simulink model "cable_driven_parallel_robot"  (R2023a)
settings: Solver=ode3  StartTime=0.0  StopTime=100  FixedStep=0.01  RelTol=1e-3
values from neighbouring files (symbols this model uses):
  cable_length = 1.2    [Model_Info.m]
  g = 9.81    [Model_Info.m]
  MP_H = 2    [Model_Info.m]
  MP_init_X = 0    [Model_Info.m]
  MP_init_Y = 0    [Model_Info.m]
  MP_init_Z = cable_length + (MP_H/2)    (= 2.2)    [Model_Info.m]
  MP_Ix = (MP_m/12)*(MP_W^2+MP_H^2)    (= 6.66666666667e-05)    [Model_Info.m]
  MP_Iy = (MP_m/12)*(MP_L^2+MP_H^2)    (= 6.66666666667e-05)    [Model_Info.m]
  MP_Iz = (MP_m/12)*(MP_L^2+MP_W^2)    (= 6.66666666667e-05)    [Model_Info.m]
  MP_L = 2    [Model_Info.m]
  MP_m = 0.0001    [Model_Info.m]
  MP_W = 2    [Model_Info.m]
  MR_init_X_L1 = -(MP_L/2)    (= -1)    [Model_Info.m]
  MR_init_X_L2 = (MP_L/2)    (= 1)    [Model_Info.m]
  MR_init_X_L3 = (MP_L/2)    (= 1)    [Model_Info.m]
  MR_init_X_L4 = -(MP_L/2)    (= -1)    [Model_Info.m]
  MR_init_Y_L1 = -(MP_W/2)    (= -1)    [Model_Info.m]
  MR_init_Y_L2 = -(MP_W/2)    (= -1)    [Model_Info.m]
  MR_init_Y_L3 = (MP_W/2)    (= 1)    [Model_Info.m]
  MR_init_Y_L4 = (MP_W/2)    (= 1)    [Model_Info.m]
  MR_init_Yaw_L1 = pi    (= 3.14159265359)    [Model_Info.m]
  MR_init_Yaw_L2 = 0    [Model_Info.m]
  MR_init_Yaw_L3 = 0    [Model_Info.m]
  MR_init_Yaw_L4 = pi    (= 3.14159265359)    [Model_Info.m]
  MR_Jr = (MR_m/12)*(MR_L^2+MR_W^2)    (= 0.333333333333)    [Model_Info.m]
  MR_m = 0.5    [Model_Info.m]
  MR_r = 2    [Model_Info.m]
  MR_WT = 2    [Model_Info.m]
  QR_Ax = 0.25*0    (= 0)    [Model_Info.m]
  QR_Ay = 0.25*0    (= 0)    [Model_Info.m]
  QR_Az = 0.25*0    (= 0)    [Model_Info.m]
  QR_b = 1.14*1e-7    (= 1.14e-07)    [Model_Info.m]
  QR_Ixx = 4.856*1e-3    (= 0.004856)    [Model_Info.m]
  QR_Iyy = 4.856*1e-3    (= 0.004856)    [Model_Info.m]
  QR_Izz = 8.801*1e-3    (= 0.008801)    [Model_Info.m]
  QR_K = 2.980*1e-6    (= 2.98e-06)    [Model_Info.m]
  QR_l = 0.225    [Model_Info.m]
  QR_m = 0.468    [Model_Info.m]
  QR_x0_U1 = -(MP_L/2)    (= -1)    [Model_Info.m]
  QR_x0_U2 = (MP_L/2)    (= 1)    [Model_Info.m]
  QR_x0_U3 = (MP_L/2)    (= 1)    [Model_Info.m]
  QR_x0_U4 = -(MP_L/2)    (= -1)    [Model_Info.m]
  QR_y0_U1 = -(MP_W/2)    (= -1)    [Model_Info.m]
  QR_y0_U2 = -(MP_W/2)    (= -1)    [Model_Info.m]
  QR_y0_U3 = (MP_W/2)    (= 1)    [Model_Info.m]
  QR_y0_U4 = (MP_W/2)    (= 1)    [Model_Info.m]
  QR_z0_U1 = 2*cable_length+(MP_H)    (= 4.4)    [Model_Info.m]
  QR_z0_U2 = 2*cable_length+(MP_H)    (= 4.4)    [Model_Info.m]
  QR_z0_U3 = 2*cable_length+(MP_H)    (= 4.4)    [Model_Info.m]
  QR_z0_U4 = 2*cable_length+(MP_H)    (= 4.4)    [Model_Info.m]
(part 10 of 12)

== matlab function cable_driven_parallel_robot/Target Wrench-Jacobian matrix/QuadRotor U1/Force Generator/QuadCopter Model ==
  data: vx input; x_ddot output size=1; vy input; vz input; phidot input; thetadot input; psidot input; y_ddot output size=1; z_ddot output size=1; phi input; theta input; psi input; constants input
function [x_ddot,y_ddot,z_ddot] = fcn(vx,vy,vz,phidot,thetadot,psidot, phi,theta,psi,constants)
m = constants(1);
g = constants(2);
Ixx = constants(3);
Iyy = constants(4);
Izz = constants(5);
l = constants(6);
K = constants(7);
b = constants(8);
Ax = constants(9);
Ay = constants(10);
Az = constants(11);
omega1 = constants(12);
omega2 = constants(13);
omega3 = constants(14);
omega4 = constants(15);
Tx = constants(16);
Ty = constants(17);
Tz = constants(18);
% x_ddot = (K*omega1^2*sin(phi)*sin(psi) - Ax*vx + K*omega2^2*sin(phi)*sin(psi) + K*omega3^2*sin(phi)*sin(psi) + K*omega4^2*sin(phi)*sin(psi) + K*omega1^2*cos(phi)*cos(psi)*sin(theta) + K*omega2^2*cos(phi)*cos(psi)*sin(theta) + K*omega3^2*cos(phi)*cos(psi)*sin(theta) + K*omega4^2*cos(phi)*cos(psi)*sin(theta))/m;
% y_ddot = -(Ay*vy + K*omega1^2*cos(psi)*sin(phi) + K*omega2^2*cos(psi)*sin(phi) + K*omega3^2*cos(psi)*sin(phi) + K*omega4^2*cos(psi)*sin(phi) - K*omega1^2*cos(phi)*sin(psi)*sin(theta) - K*omega2^2*cos(phi)*sin(psi)*sin(theta) - K*omega3^2*cos(phi)*sin(psi)*sin(theta) - K*omega4^2*cos(phi)*sin(psi)*sin(theta))/m;
% z_ddot = (K*cos(phi)*cos(theta)*omega1^2 + K*cos(phi)*cos(theta)*omega2^2 + K*cos(phi)*cos(theta)*omega3^2 + K*cos(phi)*cos(theta)*omega4^2 - Az*vz - g*m)/m;
% phi_ddot = (2*Ixx*Iyy*b*omega1^2*sin(theta) - 2*Ixx*Iyy*b*omega2^2*sin(theta) + 2*Ixx*Iyy*b*omega3^2*sin(theta) - 2*Ixx*Iyy*b*omega4^2*sin(theta) + 2*Iyy^3*psidot^2*cos(phi)*cos(theta)^4*sin(phi)^3 - 2*Iyy^3*psidot^2*cos(phi)*cos(theta)^4*sin(phi)^5 - 2*Iyy^3*psidot*thetadot*cos(theta)^3*sin(phi)^2 + 2*Iyy^3*psidot*thetadot*cos(theta)^3*sin(phi)^4 - 2*Iyy^3*psidot^2*cos(phi)^3*cos(theta)^4*sin(phi)^3 - Iyy^3*thetadot^2*sin(2*phi)*cos(theta)^2*sin(phi)^2 + Iyy^3*thetadot^2*sin(2*phi)*cos(theta)^2*sin(phi)^4 - Ixx*Iyy^2*thetadot^2*sin(2*phi)*sin(theta)^2 - 2*Iyy^2*K*l*omega2^2*cos(theta)^2*sin(phi)^2 + 2*Iyy^2*K*l*omega2^2*cos(theta)^2*sin(phi)^4 + 2*Iyy^2*K*l*omega4^2*cos(theta)^2*sin(phi)^2 - 2*Iyy^2*K*l*omega4^2*cos(theta)^2*sin(phi)^4 + 2*Ixx*Iyy^2*thetadot^2*cos(phi)*sin(phi)*sin(theta)^2 - 2*Ixx*Iyy*b*omega1^2*sin(phi)^2*sin(theta) + 2*Ixx*Iyy*b*omega2^2*sin(phi)^2*sin(theta) - 2*Ixx*Iyy*b*omega3^2*sin(phi)^2*sin(theta) + 2*Ixx*Iyy*b*omega4^2*sin(phi)^2*sin(theta) + 2*Ixx*Izz*b*omega1^2*sin(phi)^2*sin(theta) - 2*Ixx*Izz*b*omega2^2*sin(phi)^2*sin(theta) + 2*Ixx*Izz*b*omega3^2*sin(phi)^2*sin(theta) - 2*Ixx*Izz*b*omega4^2*sin(phi)^2*sin(theta) - 2*Ixx*Iyy^2*psidot*thetadot*cos(theta)*sin(theta)^2 + 2*Ixx^2*Iyy*psidot*thetadot*cos(theta)*sin(theta)^2 + 2*Ixx*Iyy^2*psidot*thetadot*sin(2*theta)*sin(theta) - 2*Ixx^2*Iyy*psidot*thetadot*sin(2*theta)*sin(theta) - 2*Iyy*Izz^2*psidot^2*cos(phi)^3*cos(theta)^4*sin(phi) - 2*Iyy^2*Izz*psidot^2*cos(phi)*cos(theta)^4*sin(phi)^3 + 2*Iyy^2*Izz*psidot^2*cos(phi)^3*cos(theta)^4*sin(phi) - 2*Iyy*Izz^2*psidot^2*cos(phi)*cos(theta)^4*sin(phi)^5 + 4*Iyy^2*Izz*psidot^2*cos(phi)*cos(theta)^4*sin(phi)^5 - 2*Ixx*Iyy^2*thetadot^2*cos(phi)*sin(phi)^3*sin(theta)^2 - 2*Ixx*Izz^2*thetadot^2*cos(phi)*sin(phi)^3*sin(theta)^2 + Ixx*Iyy*Izz*thetadot^2*sin(2*phi)*sin(theta)^2 + 6*Iyy^3*psidot*thetadot*cos(phi)^2*cos(theta)^3*sin(phi)^2 - 4*Iyy^3*psidot*thetadot*cos(phi)^2*cos(theta)^3*sin(phi)^4 - 4*Iyy^3*psidot*thetadot*cos(phi)^4*cos(theta)^3*sin(phi)^2 + 2*Iyy*Izz^2*psidot*thetadot*cos(phi)^2*cos(theta)^3 - 2*Iyy^2*Izz*psidot*thetadot*cos(phi)^2*cos(theta)^3 - 4*Iyy*Izz^2*psidot*thetadot*cos(phi)^4*cos(theta)^3 + 4*Iyy^2*Izz*psidot*thetadot*cos(phi)^4*cos(theta)^3 + 2*Ixx*Iyy^2*psidot*thetadot*cos(theta)^3*sin(phi)^2 - 2*Ixx*Iyy^2*psidot*thetadot*cos(theta)^3*sin(phi)^4 + 2*Iyy^2*Izz*psidot*thetadot*cos(theta)^3*sin(phi)^2 + 2*Iyy*Izz^2*psidot*thetadot*cos(theta)^3*sin(phi)^4 - 4*Iyy^2*Izz*psidot*thetadot*cos(theta)^3*sin(phi)^4 - 2*Ixx*Iyy*K*l*omega2^2*sin(theta)^2 + 2*Ixx*Iyy*K*l*omega4^2*sin(theta)^2 + Iyy^3*thetadot^2*sin(2*phi)*cos(phi)^2*cos(theta)^2*sin(phi)^2 - 2*Iyy*Izz^2*psidot^2*cos(phi)^3*cos(theta)^4*sin(phi)^3 + 4*Iyy^2*Izz*psidot^2*cos(phi)^3*cos(theta)^4*sin(phi)^3 + Iyy*Izz^2*thetadot^2*sin(2*phi)*cos(phi)^2*cos(theta)^2 - Iyy^2*Izz*thetadot^2*sin(2*phi)*cos(phi)^2*cos(theta)^2 + Iyy^2*Izz*thetadot^2*sin(2*phi)*cos(theta)^2*sin(phi)^2 + Iyy*Izz^2*thetadot^2*sin(2*phi)*cos(theta)^2*sin(phi)^4 - 2*Iyy^2*Izz*thetadot^2*sin(2*phi)*cos(theta)^2*sin(phi)^4 + Ixx*Iyy^2*thetadot^2*sin(2*phi)*sin(phi)^2*sin(theta)^2 + Ixx*Izz^2*thetadot^2*sin(2*phi)*sin(phi)^2*sin(theta)^2 + 2*Ixx*Iyy^2*phidot*thetadot*cos(theta)*sin(theta) + 2*Ixx^2*Iyy*phidot*thetadot*cos(theta)*sin(theta) + 2*Ixx*Iyy*K*l*omega2^2*sin(phi)^2*sin(theta)^2 - 2*Ixx*Iyy*K*l*omega4^2*sin(phi)^2*sin(theta)^2 - 2*Ixx*Izz*K*l*omega2^2*sin(phi)^2*sin(theta)^2 + 2*Ixx*Izz*K*l*omega4^2*sin(phi)^2*sin(theta)^2 - 2*Ixx*Iyy*Izz*thetadot^2*cos(phi)*sin(phi)*sin(theta)^2 + Iyy*Izz^2*thetadot^2*sin(2*phi)*cos(phi)^2*cos(theta)^2*sin(phi)^2 - 2*Iyy^2*Izz*thetadot^2*sin(2*phi)*cos(phi)^2*cos(theta)^2*sin(phi)^2 - 4*Ixx*Iyy^2*phidot*thetadot*cos(phi)^2*cos(theta)*sin(theta) - 2*Ixx*Iyy^2*phidot*thetadot*cos(theta)*sin(phi)^2*sin(theta) - 2*Ixx^2*Iyy*phidot*thetadot*cos(theta)*sin(phi)^2*sin(theta) - 2*Ixx*Izz^2*phidot*thetadot*cos(theta)*sin(phi)^2*sin(theta) + 2*Ixx^2*Izz*phidot*thetadot*cos(theta)*sin(phi)^2*sin(theta) + 2*Iyy^2*K*l*omega2^2*cos(phi)^2*cos(theta)^2*sin(phi)^2 - 2*Iyy^2*K*l*omega4^2*cos(phi)^2*cos(theta)^2*sin(phi)^2 + 2*Ixx*Iyy*Izz*psidot*thetadot*cos(theta)*sin(theta)^2 + 2*Ixx*Iyy^2*psidot^2*cos(phi)*cos(theta)^2*sin(phi)*sin(theta)^2 + 4*Ixx*Iyy*Izz*thetadot^2*cos(phi)*sin(phi)^3*sin(theta)^2 + 2*Ixx*Iyy*Izz*psidot*thetadot*cos(phi)^2*cos(theta)^3 + 2*Ixx*Iyy^2*psidot*thetadot*cos(theta)*sin(phi)^2*sin(theta)^2 - 2*Ixx^2*Iyy*psidot*thetadot*cos(theta)*sin(phi)^2*sin(theta)^2 + 2*Ixx*Izz^2*psidot*thetadot*cos(theta)*sin(phi)^2*sin(theta)^2 + 2*Ixx^2*Izz*psidot*thetadot*cos(theta)*sin(phi)^2*sin(theta)^2 + 2*Ixx*Iyy*Izz*psidot*thetadot*cos(theta)^3*sin(phi)^4 - 2*Ixx*Iyy^2*psidot*thetadot*sin(2*theta)*sin(phi)^2*sin(theta) + 2*Ixx^2*Iyy*psidot*thetadot*sin(2*theta)*sin(phi)^2*sin(theta) - 2*Ixx^2*Izz*psidot*thetadot*sin(2*theta)*sin(phi)^2*sin(theta) - 2*Ixx*Izz^2*psidot^2*cos(phi)*cos(theta)^2*sin(phi)^3*sin(theta)^2 - 2*Ixx*Izz^2*psidot^2*cos(phi)^3*cos(theta)^2*sin(phi)*sin(theta)^2 - 2*Ixx*Iyy*Izz*thetadot^2*sin(2*phi)*sin(phi)^2*sin(theta)^2 - 2*Ixx*Iyy*Izz*phidot*thetadot*cos(theta)*sin(theta) - 2*Iyy*Izz*K*l*omega2^2*cos(phi)^2*cos(theta)^2 + 2*Iyy*Izz*K*l*omega4^2*cos(phi)^2*cos(theta)^2 - 2*Ixx*Iyy^2*psidot*thetadot*cos(phi)^2*cos(theta)^3*sin(phi)^2 + 2*Iyy*Izz^2*psidot*thetadot*cos(phi)^2*cos(theta)^3*sin(phi)^2 - 8*Iyy^2*Izz*psidot*thetadot*cos(phi)^2*cos(theta)^3*sin(phi)^2 - 4*Iyy*Izz^2*psidot*thetadot*cos(phi)^2*cos(theta)^3*sin(phi)^4 - 4*Iyy*Izz^2*psidot*thetadot*cos(phi)^4*cos(theta)^3*sin(phi)^2 + 8*Iyy^2*Izz*psidot*thetadot*cos(phi)^2*cos(theta)^3*sin(phi)^4 + 8*Iyy^2*Izz*psidot*thetadot*cos(phi)^4*cos(theta)^3*sin(phi)^2 - 2*Iyy*Izz*K*l*omega2^2*cos(theta)^2*sin(phi)^4 + 2*Iyy*Izz*K*l*omega4^2*cos(theta)^2*sin(phi)^4 - 4*Ixx*Iyy^2*phidot*psidot*cos(phi)*cos(theta)^2*sin(phi)*sin(theta) + 2*Ixx^2*Iyy*phidot*psidot*cos(phi)*cos(theta)^2*sin(phi)*sin(theta) - 2*Ixx^2*Izz*phidot*psidot*cos(phi)*cos(theta)^2*sin(phi)*sin(theta) + 4*Ixx*Iyy*Izz*phidot*thetadot*cos(phi)^2*cos(theta)*sin(theta) + 4*Ixx*Iyy*Izz*phidot*thetadot*cos(theta)*sin(phi)^2*sin(theta) - 2*Iyy*Izz*K*l*omega2^2*cos(phi)^2*cos(theta)^2*sin(phi)^2 + 2*Iyy*Izz*K*l*omega4^2*cos(phi)^2*cos(theta)^2*sin(phi)^2 - 2*Ixx*Iyy*Izz*psidot^2*cos(phi)*cos(theta)^2*sin(phi)*sin(theta)^2 + 2*Ixx*Iyy^2*phidot*psidot*cos(phi)*cos(theta)^2*sin(phi)^3*sin(theta) + 2*Ixx*Iyy^2*phidot*psidot*cos(phi)^3*cos(theta)^2*sin(phi)*sin(theta) + 2*Ixx*Izz^2*phidot*psidot*cos(phi)*cos(theta)^2*sin(phi)^3*sin(theta) + 2*Ixx*Izz^2*phidot*psidot*cos(phi)^3*cos(theta)^2*sin(phi)*sin(theta) + 4*Ixx*Iyy^2*phidot*thetadot*cos(phi)^2*cos(theta)*sin(phi)^2*sin(theta) + 4*Ixx*Izz^2*phidot*thetadot*cos(phi)^2*cos(theta)*sin(phi)^2*sin(theta) - 4*Ixx*Iyy*Izz*psidot*thetadot*cos(theta)*sin(phi)^2*sin(theta)^2 + 2*Ixx*Iyy*Izz*psidot*thetadot*sin(2*theta)*sin(phi)^2*sin(theta) + 2*Ixx*Iyy*Izz*psidot^2*cos(phi)*cos(theta)^2*sin(phi)^3*sin(theta)^2 + 2*Ixx*Iyy*Izz*psidot^2*cos(phi)^3*cos(theta)^2*sin(phi)*sin(theta)^2 + 2*Ixx*Iyy*Izz*psidot*thetadot*cos(phi)^2*cos(theta)^3*sin(phi)^2 - Ixx^2*Iyy*psidot^2*sin(2*theta)*cos(phi)*cos(theta)*sin(phi)*sin(theta) + Ixx^2*Izz*psidot^2*sin(2*theta)*cos(phi)*cos(theta)*sin(phi)*sin(theta) - 4*Ixx*Iyy*Izz*phidot*psidot*cos(phi)*cos(theta)^2*sin(phi)^3*sin(theta) - 4*Ixx*Iyy*Izz*phidot*psidot*cos(phi)^3*cos(theta)^2*sin(phi)*sin(theta) - 8*Ixx*Iyy*Izz*phidot*thetadot*cos(phi)^2*cos(theta)*sin(phi)^2*sin(theta) + 2*Ixx*Iyy*K*l*omega1^2*cos(phi)*cos(theta)*sin(phi)*sin(theta) - 2*Ixx*Iyy*K*l*omega3^2*cos(phi)*cos(theta)*sin(phi)*sin(theta) - 2*Ixx*Izz*K*l*omega1^2*cos(phi)*cos(theta)*sin(phi)*sin(theta) + 2*Ixx*Izz*K*l*omega3^2*cos(phi)*cos(theta)*sin(phi)*sin(theta) - 2*Ixx*Iyy^2*phidot*thetadot*sin(2*phi)*cos(phi)*cos(theta)*sin(phi)*sin(theta) - 2*Ixx*Izz^2*phidot*thetadot*sin(2*phi)*cos(phi)*cos(theta)*sin(phi)*sin(theta) + 4*Ixx*Iyy*Izz*phidot*psidot*cos(phi)*cos(theta)^2*sin(phi)*sin(theta) + 4*Ixx*Iyy*Izz*phidot*thetadot*sin(2*phi)*cos(phi)*cos(theta)*sin(phi)*sin(theta))/(2*Ixx*cos(theta)^2*(- Iyy^2*cos(phi)^2*sin(phi)^2 - Iyy^2*sin(phi)^4 + Iyy^2*sin(phi)^2 + Izz*Iyy*cos(phi)^2*sin(phi)^2 + Izz*Iyy*cos(phi)^2 + Izz*Iyy*sin(phi)^4));
% theta_ddot = -(2*Izz^2*psidot^2*cos(phi)^4*cos(theta)^2*sin(theta) + 2*Iyy^2*thetadot^2*cos(phi)^2*sin(phi)^2*sin(theta) + 2*Izz^2*thetadot^2*cos(phi)^2*sin(phi)^2*sin(theta) + 2*Iyy^2*psidot^2*cos(theta)^2*sin(phi)^4*sin(theta) - 2*Izz^2*phidot*psidot*cos(phi)^4*cos(theta)^2 - 2*Iyy^2*phidot*psidot*cos(theta)^2*sin(phi)^4 + 2*Iyy*b*omega1^2*cos(phi)*sin(phi) - 2*Iyy*b*omega2^2*cos(phi)*sin(phi) + 2*Iyy*b*omega3^2*cos(phi)*sin(phi) - 2*Iyy*b*omega4^2*cos(phi)*sin(phi) - 2*Izz*b*omega1^2*cos(phi)*sin(phi) + 2*Izz*b*omega2^2*cos(phi)*sin(phi) - 2*Izz*b*omega3^2*cos(phi)*sin(phi) + 2*Izz*b*omega4^2*cos(phi)*sin(phi) - Ixx*Izz*psidot^2*sin(2*theta)*cos(phi)^2*cos(theta) - 4*Iyy*Izz*thetadot^2*cos(phi)^2*sin(phi)^2*sin(theta) - Ixx*Iyy*psidot^2*sin(2*theta)*cos(theta)*sin(phi)^2 + 2*Izz*K*l*omega1^2*cos(phi)^2*cos(theta) - 2*Izz*K*l*omega3^2*cos(phi)^2*cos(theta) + 2*Izz^2*phidot*thetadot*sin(2*phi)*cos(phi)^2*cos(theta) + 2*Ixx*Izz*phidot*psidot*cos(phi)^2*cos(theta)^2 + 2*Iyy*Izz*phidot*psidot*cos(phi)^4*cos(theta)^2 + 2*Iyy*K*l*omega1^2*cos(theta)*sin(phi)^2 - 2*Iyy*K*l*omega3^2*cos(theta)*sin(phi)^2 - 2*Iyy^2*phidot*thetadot*sin(2*phi)*cos(theta)*sin(phi)^2 + 2*Ixx*Iyy*phidot*psidot*cos(theta)^2*sin(phi)^2 + 2*Iyy*Izz*phidot*psidot*cos(theta)^2*sin(phi)^4 + 2*Iyy^2*psidot^2*cos(phi)^2*cos(theta)^2*sin(phi)^2*sin(theta) + 2*Izz^2*psidot^2*cos(phi)^2*cos(theta)^2*sin(phi)^2*sin(theta) + 2*Iyy^2*phidot*thetadot*cos(phi)*cos(theta)*sin(phi) + 2*Izz^2*phidot*thetadot*cos(phi)*cos(theta)*sin(phi) - 2*Iyy^2*phidot*psidot*cos(phi)^2*cos(theta)^2*sin(phi)^2 - 2*Izz^2*phidot*psidot*cos(phi)^2*cos(theta)^2*sin(phi)^2 - Iyy^2*thetadot^2*sin(2*phi)*cos(phi)*sin(phi)*sin(theta) - Izz^2*thetadot^2*sin(2*phi)*cos(phi)*sin(phi)*sin(theta) - 4*Iyy^2*phidot*thetadot*cos(phi)^3*cos(theta)*sin(phi) - 4*Izz^2*phidot*thetadot*cos(phi)^3*cos(theta)*sin(phi) + 2*Iyy^2*psidot*thetadot*sin(2*theta)*cos(phi)*sin(phi) - 2*Iyy*Izz*phidot*thetadot*sin(2*phi)*cos(phi)^2*cos(theta) + 2*Iyy*Izz*phidot*thetadot*sin(2*phi)*cos(theta)*sin(phi)^2 - 2*Iyy^2*psidot*thetadot*cos(phi)*cos(theta)*sin(phi)*sin(theta) - 2*Izz^2*psidot*thetadot*cos(phi)*cos(theta)*sin(phi)*sin(theta) + 2*Ixx*Iyy*phidot*thetadot*cos(phi)*cos(theta)*sin(phi) - 2*Ixx*Izz*phidot*thetadot*cos(phi)*cos(theta)*sin(phi) - 4*Iyy*Izz*phidot*thetadot*cos(phi)*cos(theta)*sin(phi) + 4*Iyy*Izz*phidot*psidot*cos(phi)^2*cos(theta)^2*sin(phi)^2 + 2*Iyy*Izz*thetadot^2*sin(2*phi)*cos(phi)*sin(phi)*sin(theta) + 8*Iyy*Izz*phidot*thetadot*cos(phi)^3*cos(theta)*sin(phi) - 2*Iyy*K*l*omega2^2*cos(phi)*sin(phi)*sin(theta) + 2*Iyy*K*l*omega4^2*cos(phi)*sin(phi)*sin(theta) + 2*Izz*K*l*omega2^2*cos(phi)*sin(phi)*sin(theta) - 2*Izz*K*l*omega4^2*cos(phi)*sin(phi)*sin(theta) - 2*Ixx*Iyy*psidot*thetadot*sin(2*theta)*cos(phi)*sin(phi) + 2*Ixx*Izz*psidot*thetadot*sin(2*theta)*cos(phi)*sin(phi) - 2*Iyy*Izz*psidot*thetadot*sin(2*theta)*cos(phi)*sin(phi) + 2*Ixx*Iyy*psidot*thetadot*cos(phi)*cos(theta)*sin(phi)*sin(theta) - 2*Ixx*Izz*psidot*thetadot*cos(phi)*cos(theta)*sin(phi)*sin(theta) + 4*Iyy*Izz*psidot*thetadot*cos(phi)*cos(theta)*sin(phi)*sin(theta))/(2*cos(theta)*(- Iyy^2*cos(phi)^2*sin(phi)^2 - Iyy^2*sin(phi)^4 + Iyy^2*sin(phi)^2 + Izz*Iyy*cos(phi)^2*sin(phi)^2 + Izz*Iyy*cos(phi)^2 + Izz*Iyy*sin(phi)^4));
% psi_ddot = (2*Iyy*b*omega1^2 - 2*Iyy*b*omega2^2 + 2*Iyy*b*omega3^2 - 2*Iyy*b*omega4^2 - Iyy^2*thetadot^2*sin(2*phi)*sin(theta) - 2*Iyy*b*omega1^2*sin(phi)^2 + 2*Iyy*b*omega2^2*sin(phi)^2 - 2*Iyy*b*omega3^2*sin(phi)^2 + 2*Iyy*b*omega4^2*sin(phi)^2 + 2*Izz*b*omega1^2*sin(phi)^2 - 2*Izz*b*omega2^2*sin(phi)^2 + 2*Izz*b*omega3^2*sin(phi)^2 - 2*Izz*b*omega4^2*sin(phi)^2 + 2*Iyy^2*psidot*thetadot*sin(2*theta) + 2*Iyy^2*phidot*thetadot*cos(theta) - 2*Iyy^2*phidot*thetadot*cos(theta)*sin(phi)^2 - 2*Izz^2*phidot*thetadot*cos(theta)*sin(phi)^2 - 2*Iyy*K*l*omega2^2*sin(theta) + 2*Iyy*K*l*omega4^2*sin(theta) - 2*Ixx*Iyy*psidot*thetadot*sin(2*theta) + Iyy^2*thetadot^2*sin(2*phi)*sin(phi)^2*sin(theta) + Izz^2*thetadot^2*sin(2*phi)*sin(phi)^2*sin(theta) - 2*Iyy^2*psidot*thetadot*sin(2*theta)*sin(phi)^2 + 2*Iyy^2*thetadot^2*cos(phi)*sin(phi)*sin(theta) - 2*Iyy^2*psidot*thetadot*cos(theta)*sin(theta) + 2*Ixx*Iyy*phidot*thetadot*cos(theta) - 2*Iyy*Izz*phidot*thetadot*cos(theta) - 2*Iyy^2*thetadot^2*cos(phi)*sin(phi)^3*sin(theta) - 2*Izz^2*thetadot^2*cos(phi)*sin(phi)^3*sin(theta) + Iyy*Izz*thetadot^2*sin(2*phi)*sin(theta) - 4*Iyy^2*phidot*thetadot*cos(phi)^2*cos(theta) - 2*Izz^2*psidot^2*cos(phi)*cos(theta)^2*sin(phi)^3*sin(theta) - 2*Izz^2*psidot^2*cos(phi)^3*cos(theta)^2*sin(phi)*sin(theta) - 2*Iyy*Izz*thetadot^2*sin(2*phi)*sin(phi)^2*sin(theta) + 2*Iyy^2*phidot*psidot*cos(phi)*cos(theta)^2*sin(phi)^3 + 2*Iyy^2*phidot*psidot*cos(phi)^3*cos(theta)^2*sin(phi) + 2*Izz^2*phidot*psidot*cos(phi)*cos(theta)^2*sin(phi)^3 + 2*Izz^2*phidot*psidot*cos(phi)^3*cos(theta)^2*sin(phi) + 4*Iyy^2*phidot*thetadot*cos(phi)^2*cos(theta)*sin(phi)^2 + 4*Izz^2*phidot*thetadot*cos(phi)^2*cos(theta)*sin(phi)^2 + 2*Iyy*K*l*omega2^2*sin(phi)^2*sin(theta) - 2*Iyy*K*l*omega4^2*sin(phi)^2*sin(theta) - 2*Izz*K*l*omega2^2*sin(phi)^2*sin(theta) + 2*Izz*K*l*omega4^2*sin(phi)^2*sin(theta) + 2*Ixx*Iyy*psidot*thetadot*sin(2*theta)*sin(phi)^2 - 2*Ixx*Izz*psidot*thetadot*sin(2*theta)*sin(phi)^2 + 2*Iyy*Izz*psidot*thetadot*sin(2*theta)*sin(phi)^2 - 2*Iyy*Izz*thetadot^2*cos(phi)*sin(phi)*sin(theta) + 2*Ixx*Iyy*psidot*thetadot*cos(theta)*sin(theta) + 2*Iyy*Izz*psidot*thetadot*cos(theta)*sin(theta) + 2*Iyy^2*psidot^2*cos(phi)*cos(theta)^2*sin(phi)*sin(theta) + 4*Iyy*Izz*thetadot^2*cos(phi)*sin(phi)^3*sin(theta) - 4*Iyy^2*phidot*psidot*cos(phi)*cos(theta)^2*sin(phi) + 4*Iyy*Izz*phidot*thetadot*cos(phi)^2*cos(theta) + 2*Iyy^2*psidot*thetadot*cos(theta)*sin(phi)^2*sin(theta) + 2*Izz^2*psidot*thetadot*cos(theta)*sin(phi)^2*sin(theta) - 2*Ixx*Iyy*phidot*thetadot*cos(theta)*sin(phi)^2 + 2*Ixx*Izz*phidot*thetadot*cos(theta)*sin(phi)^2 + 4*Iyy*Izz*phidot*thetadot*cos(theta)*sin(phi)^2 - 4*Iyy*Izz*phidot*psidot*cos(phi)*cos(theta)^2*sin(phi)^3 - 4*Iyy*Izz*phidot*psidot*cos(phi)^3*cos(theta)^2*sin(phi) - 8*Iyy*Izz*phidot*thetadot*cos(phi)^2*cos(theta)*sin(phi)^2 - Ixx*Iyy*psidot^2*sin(2*theta)*cos(phi)*cos(theta)*sin(phi) + Ixx*Izz*psidot^2*sin(2*theta)*cos(phi)*cos(theta)*sin(phi) - 2*Iyy*Izz*psidot^2*cos(phi)*cos(theta)^2*sin(phi)*sin(theta) + 2*Iyy*K*l*omega1^2*cos(phi)*cos(theta)*sin(phi) - 2*Iyy*K*l*omega3^2*cos(phi)*cos(theta)*sin(phi) - 2*Izz*K*l*omega1^2*cos(phi)*cos(theta)*sin(phi) + 2*Izz*K*l*omega3^2*cos(phi)*cos(theta)*sin(phi) - 2*Iyy^2*phidot*thetadot*sin(2*phi)*cos(phi)*cos(theta)*sin(phi) - 2*Izz^2*phidot*thetadot*sin(2*phi)*cos(phi)*cos(theta)*sin(phi) + 2*Ixx*Iyy*phidot*psidot*cos(phi)*cos(theta)^2*sin(phi) - 2*Ixx*Izz*phidot*psidot*cos(phi)*cos(theta)^2*sin(phi) + 4*Iyy*Izz*phidot*psidot*cos(phi)*cos(theta)^2*sin(phi) - 2*Ixx*Iyy*psidot*thetadot*cos(theta)*sin(phi)^2*sin(theta) + 2*Ixx*Izz*psidot*thetadot*cos(theta)*sin(phi)^2*sin(theta) - 4*Iyy*Izz*psidot*thetadot*cos(theta)*sin(phi)^2*sin(theta) + 2*Iyy*Izz*psidot^2*cos(phi)*cos(theta)^2*sin(phi)^3*sin(theta) + 2*Iyy*Izz*psidot^2*cos(phi)^3*cos(theta)^2*sin(phi)*sin(theta) + 4*Iyy*Izz*phidot*thetadot*sin(2*phi)*cos(phi)*cos(theta)*sin(phi))/(2*cos(theta)^2*(- Iyy^2*cos(phi)^2*sin(phi)^2 - Iyy^2*sin(phi)^4 + Iyy^2*sin(phi)^2 + Izz*Iyy*cos(phi)^2*sin(phi)^2 + Izz*Iyy*cos(phi)^2 + Izz*Iyy*sin(phi)^4));
x_ddot =  (K*omega1^2*sin(phi)*sin(psi) - Ax*vx - Tx + K*omega2^2*sin(phi)*sin(psi) + K*omega3^2*sin(phi)*sin(psi) + K*omega4^2*sin(phi)*sin(psi) + K*omega1^2*cos(phi)*cos(psi)*sin(theta) + K*omega2^2*cos(phi)*cos(psi)*sin(theta) + K*omega3^2*cos(phi)*cos(psi)*sin(theta) + K*omega4^2*cos(phi)*cos(psi)*sin(theta))/m;
y_ddot = -(Ty + Ay*vy + K*omega1^2*cos(psi)*sin(phi) + K*omega2^2*cos(psi)*sin(phi) + K*omega3^2*cos(psi)*sin(phi) + K*omega4^2*cos(psi)*sin(phi) - K*omega1^2*cos(phi)*sin(psi)*sin(theta) - K*omega2^2*cos(phi)*sin(psi)*sin(theta) - K*omega3^2*cos(phi)*sin(psi)*sin(theta) - K*omega4^2*cos(phi)*sin(psi)*sin(theta))/m;
z_ddot = (K*cos(phi)*cos(theta)*omega1^2 + K*cos(phi)*cos(theta)*omega2^2 + K*cos(phi)*cos(theta)*omega3^2 + K*cos(phi)*cos(theta)*omega4^2 - Tz - Az*vz - g*m)/m;

end

== matlab function cable_driven_parallel_robot/Target Wrench-Jacobian matrix/QuadRotor U1/Force Generator/QR Force Generator ==
  data: x_rotor input; Fx output; y_rotor input; z_rotor input; x_point input; y_point input; z_point input; ax input; ay input; az input; mass input; cable_length input; Fy output; Fz output; isTension output
function [Fx,Fy,Fz,isTension] = fcn(x_rotor,y_rotor,z_rotor,x_point,y_point,z_point,ax,ay,az,mass,cable_length)
isTension =1;
distance =  sqrt((x_rotor-x_point).^2 +...
                 (y_rotor-y_point).^2 +...
                 (z_rotor-z_point).^2);
if distance < (cable_length-0.1)
   Fx = 0;
   Fy = 0;
   Fz = 0;
   isTension =0;
else
   Fx = mass*ax;
   Fy = mass*ay;
   Fz = mass*az; 
    
end
end

== matlab function cable_driven_parallel_robot/Target Wrench-Jacobian matrix/2 Wheels Diffrential Mobile Robot L1/2 Wheels Diffrential Mobile Robot/2 Wheels Diffrential Mobile Robot ==
  settings: updateMethod=DISCRETE
  data: TR input; TL input; Tx input; Tz input; mr input; r input; ax output; az output
function [ax,az] = fcn(TR,TL,Tx,Tz,mr,r)


g=9.81;

ax = ((TR/r)+(TL/r)+Tx)/mr;

az = (Tz -mr*g)/mr;

== matlab function cable_driven_parallel_robot/Target Wrench-Jacobian matrix/2 Wheels Diffrential Mobile Robot L1/2 Wheels Diffrential Mobile Robot/2 Wheels Diffrential Mobile Robot Transformation to Global ==
  settings: updateMethod=DISCRETE
  data: Ax input; Az input; yaw input; Abx output; Aby output; Abz output
function [Abx,Aby,Abz] = fcn(Ax,Az,yaw)

a=[Ax;0;Az];

R_z = [cos(yaw) -sin(yaw)  0; ...
       sin(yaw)  cos(yaw)  0; ...
       0           0       1]; 

Acc=R_z*a;

Abx = Acc(1);

Aby = Acc(2);

Abz = Acc(3);

== matlab function cable_driven_parallel_robot/Target Wrench-Jacobian matrix/2 Wheels Diffrential Mobile Robot L1/2 Wheels Diffrential Mobile Robot/QR Force Generator ==
  data: x_diff input; Fx output; y_diff input; z_diff input; x_point input; y_point input; z_point input; ax input; ay input; az input; mass input; cable_length input; Fy output; Fz output; isTension output
function [Fx,Fy,Fz,isTension] = fcn(x_diff,y_diff,z_diff,x_point,y_point,z_point,ax,ay,az,mass,cable_length)

isTension= 1;
distance =  sqrt((x_diff-x_point).^2 +...
                 (y_diff-y_point).^2 +...
                 (z_diff-z_point).^2);
if distance < (cable_length-0.1)
   Fx = 0;
   Fy = 0;
   Fz = 0;
   isTension= 0;
else
   Fx = mass*ax;
   Fy = mass*ay;
   Fz = mass*az; 
    
end
end

== matlab function cable_driven_parallel_robot/Target Wrench-Jacobian matrix/2 Wheels Diffrential Mobile Robot L2/2 Wheels Diffrential Mobile Robot/2 Wheels Diffrential Mobile Robot ==
  settings: updateMethod=DISCRETE
  data: TR input; TL input; Tx input; Tz input; mr input; r input; ax output; az output
function [ax,az] = fcn(TR,TL,Tx,Tz,mr,r)


g=9.81;

ax = ((TR/r)+(TL/r)+Tx)/mr;

az = (Tz -mr*g)/mr;

== matlab function cable_driven_parallel_robot/Target Wrench-Jacobian matrix/2 Wheels Diffrential Mobile Robot L2/2 Wheels Diffrential Mobile Robot/2 Wheels Diffrential Mobile Robot Transformation to Global ==
  settings: updateMethod=DISCRETE
  data: Ax input; Az input; yaw input; Abx output; Aby output; Abz output
function [Abx,Aby,Abz] = fcn(Ax,Az,yaw)

a=[Ax;0;Az];

R_z = [cos(yaw) -sin(yaw)  0; ...
       sin(yaw)  cos(yaw)  0; ...
       0           0       1]; 

Acc=R_z*a;

Abx = Acc(1);

Aby = Acc(2);

Abz = Acc(3);

== matlab function cable_driven_parallel_robot/Target Wrench-Jacobian matrix/2 Wheels Diffrential Mobile Robot L2/2 Wheels Diffrential Mobile Robot/QR Force Generator ==
  data: x_diff input; Fx output; y_diff input; z_diff input; x_point input; y_point input; z_point input; ax input; ay input; az input; mass input; cable_length input; Fy output; Fz output; isTension output
function [Fx,Fy,Fz,isTension] = fcn(x_diff,y_diff,z_diff,x_point,y_point,z_point,ax,ay,az,mass,cable_length)

isTension= 1;
distance =  sqrt((x_diff-x_point).^2 +...
                 (y_diff-y_point).^2 +...
                 (z_diff-z_point).^2);
if distance < (cable_length-0.1)
   Fx = 0;
   Fy = 0;
   Fz = 0;
   isTension= 0;
else
   Fx = mass*ax;
   Fy = mass*ay;
   Fz = mass*az; 
    
end
end

== matlab function cable_driven_parallel_robot/Target Wrench-Jacobian matrix/Subsystem/MATLAB Function ==
  data: QR_Fx_U1 input; QR_Tx_U1 output; QR_Fx_U2 input; QR_Fx_U3 input; QR_Fx_U4 input; MP_Fx input; MR_Fx_L1 input; MR_Fx_L2 input; MR_Fx_L3 input; MR_Fx_L4 input; isTension input; QR_x_U1 input; QR_x_U2 input; QR_x_U3 input; QR_x_U4 input; MP_U1 input; MP_U2 input; MP_U3 input; MP_U4 input; MP_L1 input; MP_L2 input; MP_L3 input; MP_L4 input; MR_x_L1 input; MR_x_L2 input; MR_x_L3 input; MR_x_L4 input; QR_m input; MP_m input; MR_m input; QR_Tx_U2 output; QR_Tx_U3 output; QR_Tx_U4 output; MR_Tx_L1 output; MR_Tx_L2 output; MR_Tx_L3 output; MR_Tx_L4 output
function [QR_Tx_U1,QR_Tx_U2,QR_Tx_U3,QR_Tx_U4,MR_Tx_L1,MR_Tx_L2,MR_Tx_L3,MR_Tx_L4] = fcn(QR_Fx_U1,QR_Fx_U2,QR_Fx_U3,QR_Fx_U4,MP_Fx,MR_Fx_L1,MR_Fx_L2,MR_Fx_L3,MR_Fx_L4,isTension,QR_x_U1,QR_x_U2,QR_x_U3,QR_x_U4,MP_U1,MP_U2,MP_U3,MP_U4,MP_L1,MP_L2,MP_L3,MP_L4,MR_x_L1,MR_x_L2,MR_x_L3,MR_x_L4,QR_m,MP_m,MR_m)

MP_Fx = MP_Fx*or(sum(isTension),0);

Fx_Total = QR_Fx_U1+QR_Fx_U2+QR_Fx_U3+QR_Fx_U4+MP_Fx+MR_Fx_L1+MR_Fx_L2+MR_Fx_L3+MR_Fx_L4;

if Fx_Total==0
    ax = 0
else

    m_Total = (isTension(1)+isTension(2)+isTension(3)+isTension(4))*QR_m +...
                                             (or(sum(isTension),0))*MP_m +...
              (isTension(5)+isTension(6)+isTension(7)+isTension(8))*MR_m;
      
    ax = Fx_Total/m_Total;
end
     
QR_Tx_U1 = max(((MP_U1(1)-QR_x_U1)/(abs(MP_U1(1)-QR_x_U1)))*(QR_m*ax - QR_Fx_U1),0)*isTension(1)
QR_Tx_U2 = max(((MP_U2(1)-QR_x_U2)/(abs(MP_U2(1)-QR_x_U2)))*(QR_m*ax - QR_Fx_U2),0)*isTension(2)
QR_Tx_U3 = max(((MP_U3(1)-QR_x_U3)/(abs(MP_U3(1)-QR_x_U3)))*(QR_m*ax - QR_Fx_U3),0)*isTension(3)
QR_Tx_U4 = max(((MP_U4(1)-QR_x_U4)/(abs(MP_U4(1)-QR_x_U4)))*(QR_m*ax - QR_Fx_U4),0)*isTension(4)
MR_Tx_L1 = max(((MP_L1(1)-MR_x_L1)/(abs(MP_L1(1)-MR_x_L1)))*(MR_m*ax - MR_Fx_L1),0)*isTension(5)
MR_Tx_L2 = max(((MP_L2(1)-MR_x_L2)/(abs(MP_L2(1)-MR_x_L2)))*(MR_m*ax - MR_Fx_L2),0)*isTension(6)
MR_Tx_L3 = max(((MP_L3(1)-MR_x_L3)/(abs(MP_L3(1)-MR_x_L3)))*(MR_m*ax - MR_Fx_L3),0)*isTension(7)
MR_Tx_L4 = max(((MP_L4(1)-MR_x_L4)/(abs(MP_L4(1)-MR_x_L4)))*(MR_m*ax - MR_Fx_L4),0)*isTension(8)


end

== matlab function cable_driven_parallel_robot/Target Wrench-Jacobian matrix/Subsystem/MATLAB Function1 ==
  data: QR_Fy_U1 input; QR_Ty_U1 output; QR_Fy_U2 input; QR_Fy_U3 input; QR_Fy_U4 input; MP_Fy input; MR_Fy_L1 input; MR_Fy_L2 input; MR_Fy_L3 input; MR_Fy_L4 input; isTension input; QR_y_U1 input; QR_y_U2 input; QR_y_U3 input; QR_y_U4 input; MP_U1 input; MP_U2 input; MP_U3 input; MP_U4 input; MP_L1 input; MP_L2 input; MP_L3 input; MP_L4 input; MR_y_L1 input; MR_y_L2 input; MR_y_L3 input; MR_y_L4 input; QR_m input; MP_m input; MR_m input; QR_Ty_U2 output; QR_Ty_U3 output; QR_Ty_U4 output; MR_Ty_L1 output; MR_Ty_L2 output; MR_Ty_L3 output; MR_Ty_L4 output
function [QR_Ty_U1,QR_Ty_U2,QR_Ty_U3, QR_Ty_U4,MR_Ty_L1,MR_Ty_L2,MR_Ty_L3,MR_Ty_L4] = fcn(QR_Fy_U1,QR_Fy_U2,QR_Fy_U3,QR_Fy_U4,MP_Fy,MR_Fy_L1,MR_Fy_L2,MR_Fy_L3,MR_Fy_L4,isTension,QR_y_U1,QR_y_U2,QR_y_U3,QR_y_U4,MP_U1,MP_U2,MP_U3,MP_U4,MP_L1,MP_L2,MP_L3,MP_L4,MR_y_L1,MR_y_L2,MR_y_L3,MR_y_L4,QR_m,MP_m,MR_m)

MP_Fy = MP_Fy*or(sum(isTension),0);

Fy_Total = QR_Fy_U1+QR_Fy_U2+QR_Fy_U3+QR_Fy_U4+MP_Fy+MR_Fy_L1+MR_Fy_L2+MR_Fy_L3+MR_Fy_L4;

if Fy_Total==0
    ay = 0;
else

    m_Total = (isTension(1)+isTension(2)+isTension(3)+isTension(4))*QR_m +...
                                             (or(sum(isTension),0))*MP_m +...
              (isTension(5)+isTension(6)+isTension(7)+isTension(8))*MR_m;
      
    ay = Fy_Total/m_Total;
end
     
QR_Ty_U1 = max(((MP_U1(2)-QR_y_U1)/(abs(MP_U1(2)-QR_y_U1)))*(QR_m*ay - QR_Fy_U1),0)*isTension(1);
QR_Ty_U2 = max(((MP_U2(2)-QR_y_U2)/(abs(MP_U2(2)-QR_y_U2)))*(QR_m*ay - QR_Fy_U2),0)*isTension(2);
QR_Ty_U3 = max(((MP_U3(2)-QR_y_U3)/(abs(MP_U3(2)-QR_y_U3)))*(QR_m*ay - QR_Fy_U3),0)*isTension(3);
QR_Ty_U4 = max(((MP_U4(2)-QR_y_U4)/(abs(MP_U4(2)-QR_y_U4)))*(QR_m*ay - QR_Fy_U4),0)*isTension(4);
MR_Ty_L1 = max(((MP_L1(2)-MR_y_L1)/(abs(MP_L1(2)-MR_y_L1)))*(MR_m*ay - MR_Fy_L1),0)*isTension(5);
MR_Ty_L2 = max(((MP_L2(2)-MR_y_L2)/(abs(MP_L2(2)-MR_y_L2)))*(MR_m*ay - MR_Fy_L2),0)*isTension(6);
MR_Ty_L3 = max(((MP_L3(2)-MR_y_L3)/(abs(MP_L3(2)-MR_y_L3)))*(MR_m*ay - MR_Fy_L3),0)*isTension(7);
MR_Ty_L4 = max(((MP_L4(2)-MR_y_L4)/(abs(MP_L4(2)-MR_y_L4)))*(MR_m*ay - MR_Fy_L4),0)*isTension(8);


end

== matlab function cable_driven_parallel_robot/Target Wrench-Jacobian matrix/2 Wheels Diffrential Mobile Robot L3/2 Wheels Diffrential Mobile Robot/2 Wheels Diffrential Mobile Robot ==
  settings: updateMethod=DISCRETE
  data: TR input; TL input; Tx input; Tz input; mr input; r input; ax output; az output
function [ax,az] = fcn(TR,TL,Tx,Tz,mr,r)


g=9.81;

ax = ((TR/r)+(TL/r)+Tx)/mr;

az = (Tz -mr*g)/mr;

== matlab function cable_driven_parallel_robot/Target Wrench-Jacobian matrix/2 Wheels Diffrential Mobile Robot L3/2 Wheels Diffrential Mobile Robot/2 Wheels Diffrential Mobile Robot Transformation to Global ==
  settings: updateMethod=DISCRETE
  data: Ax input; Az input; yaw input; Abx output; Aby output; Abz output
function [Abx,Aby,Abz] = fcn(Ax,Az,yaw)

a=[Ax;0;Az];

R_z = [cos(yaw) -sin(yaw)  0; ...
       sin(yaw)  cos(yaw)  0; ...
       0           0       1]; 

Acc=R_z*a;

Abx = Acc(1);

Aby = Acc(2);

Abz = Acc(3);

== matlab function cable_driven_parallel_robot/Target Wrench-Jacobian matrix/2 Wheels Diffrential Mobile Robot L3/2 Wheels Diffrential Mobile Robot/QR Force Generator ==
  data: x_diff input; Fx output; y_diff input; z_diff input; x_point input; y_point input; z_point input; ax input; ay input; az input; mass input; cable_length input; Fy output; Fz output; isTension output
function [Fx,Fy,Fz,isTension] = fcn(x_diff,y_diff,z_diff,x_point,y_point,z_point,ax,ay,az,mass,cable_length)

isTension= 1;
distance =  sqrt((x_diff-x_point).^2 +...
                 (y_diff-y_point).^2 +...
                 (z_diff-z_point).^2);
if distance < (cable_length-0.1)
   Fx = 0;
   Fy = 0;
   Fz = 0;
   isTension= 0;
else
   Fx = mass*ax;
   Fy = mass*ay;
   Fz = mass*az; 
    
end
end

== matlab function cable_driven_parallel_robot/Target Wrench-Jacobian matrix/2 Wheels Diffrential Mobile Robot L4/2 Wheels Diffrential Mobile Robot/2 Wheels Diffrential Mobile Robot ==
  settings: updateMethod=DISCRETE
  data: TR input; TL input; Tx input; Tz input; mr input; r input; ax output; az output
function [ax,az] = fcn(TR,TL,Tx,Tz,mr,r)


g=9.81;

ax = ((TR/r)+(TL/r)+Tx)/mr;

az = (Tz -mr*g)/mr;

== matlab function cable_driven_parallel_robot/Target Wrench-Jacobian matrix/2 Wheels Diffrential Mobile Robot L4/2 Wheels Diffrential Mobile Robot/2 Wheels Diffrential Mobile Robot Transformation to Global ==
  settings: updateMethod=DISCRETE
  data: Ax input; Az input; yaw input; Abx output; Aby output; Abz output
function [Abx,Aby,Abz] = fcn(Ax,Az,yaw)

a=[Ax;0;Az];

R_z = [cos(yaw) -sin(yaw)  0; ...
       sin(yaw)  cos(yaw)  0; ...
       0           0       1]; 

Acc=R_z*a;

Abx = Acc(1);

Aby = Acc(2);

Abz = Acc(3);

== matlab function cable_driven_parallel_robot/Target Wrench-Jacobian matrix/2 Wheels Diffrential Mobile Robot L4/2 Wheels Diffrential Mobile Robot/QR Force Generator ==
  data: x_diff input; Fx output; y_diff input; z_diff input; x_point input; y_point input; z_point input; ax input; ay input; az input; mass input; cable_length input; Fy output; Fz output; isTension output
function [Fx,Fy,Fz,isTension] = fcn(x_diff,y_diff,z_diff,x_point,y_point,z_point,ax,ay,az,mass,cable_length)

isTension= 1;
distance =  sqrt((x_diff-x_point).^2 +...
                 (y_diff-y_point).^2 +...
                 (z_diff-z_point).^2);
if distance < (cable_length-0.1)
   Fx = 0;
   Fy = 0;
   Fz = 0;
   isTension= 0;
else
   Fx = mass*ax;
   Fy = mass*ay;
   Fz = mass*az; 
    
end
end

== matlab function cable_driven_parallel_robot/Target Wrench-Jacobian matrix/QuadRotor U2/Force Generator/QR Force Generator ==
  data: x_rotor input; Fx output; y_rotor input; z_rotor input; x_point input; y_point input; z_point input; ax input; ay input; az input; mass input; cable_length input; Fy output; Fz output; isTension output
function [Fx,Fy,Fz,isTension] = fcn(x_rotor,y_rotor,z_rotor,x_point,y_point,z_point,ax,ay,az,mass,cable_length)
isTension =1;
distance =  sqrt((x_rotor-x_point).^2 +...
                 (y_rotor-y_point).^2 +...
                 (z_rotor-z_point).^2);
if distance < (cable_length-0.1)
   Fx = 0;
   Fy = 0;
   Fz = 0;
   isTension =0;
else
   Fx = mass*ax;
   Fy = mass*ay;
   Fz = mass*az; 
    
end
end
